simulink model "gtm_design"  (R2021b)
settings: Solver=VariableStepAuto  StartTime=0.0  StopTime=30  MinStep=0.0049  RelTol=1e-3
StopFcn:
  | MWSout=grabmws(bdroot);
  | MWSout.lastrun=datestr(now);
values from neighbouring files (symbols this model uses):
  g = 32.17405    [SingleDOF.m]    (also in layer1atm.m; mainSimple.m = 32.174; simio.m = [dx(Index.EOM(1:6)); delta(:)-f; -delta(:)-f ])
  GuidanceMode = 1    [mainSimple.m]    (also in setup.m)
  knots2fps = 1/fps2knots    (= 1.687800745)    [main.m]    (also in mainSimple.m = 1.68781)
  s = tf('s')    [SingleDOF.m]    (also in main.m; mainSimple.m; newmain.m)
undefined symbols (not defined in the file or in its folder): Aero, aftfuel, aftfuel_pos, AILL, AILLC, AILR, AILRC, alpha_deg, altitude_ft, Ax_g, Ay_g, Az_g, b, beta_deg, bias, BRAKEC, Cbar, cg_pos0, cg_shift_gear, DamageCase, DamageModels, DamageOnsetTime, Earth, ELLIB, ELLIBC, ELLOB, ELLOBC, ELRIB, ELRIBC, ELROB, ELROBC, engl_ang, engl_pos, engr_ang, engr_pos, FLAPLC, FLAPLIB, FLAPLOB, FLAPRC, FLAPRIB, FLAPROB, FuelUsed_Init, fwdfuel, fwdfuel_pos, GEAR, GEARC, Inertia0, Inertia_shift_gear, Ixx_model, Iyy_model, Izz_model, KTAS, LandingGear, LengON, LinearizeModeOn, m, MORPHLC, MORPHRC, NAV_altitude_m, NAV_latitude_deg ... (+51)
libraries: simulink_extras x39, simulink_need_slupdate x30, LPVBlockLibrary x9, aerolibconvert2 x7, simulink x3, aerolibtransform2 x3, UserContent_lib x2, uavalgslib x2, robotcorelib x1, uavutilslib x1
(part 5 of 7)

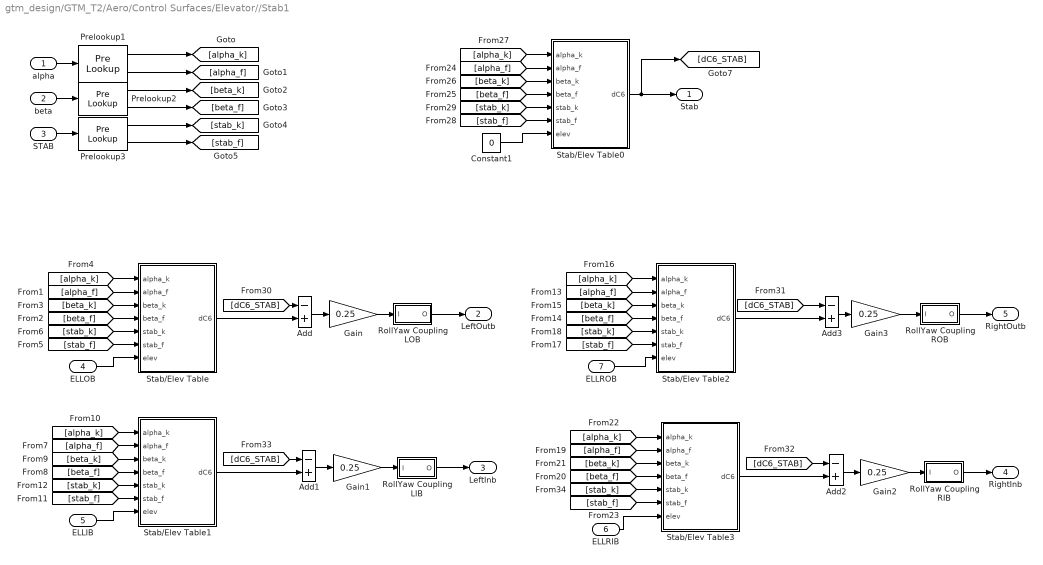
== system gtm_design/GTM_T2/Aero/Control Surfaces/Elevator//Stab1 ==
  alpha : Inport
  beta : Inport  Port=2
  STAB : Inport  Port=3
  ELLOB : Inport  Port=4
  ELLIB : Inport  Port=5
  ELLRIB : Inport  Port=6
  ELLROB : Inport  Port=7
  Add{,1..3} (4 alike) : Sum  Inputs=-+
  Constant1 : Constant  Value=0
  Gain{,1..3} (4 alike) : Gain  Gain=0.25
  Prelookup1 : PreLookup  BreakpointsData=Aero.dC3_ele.alpha  IndexSearchMethod=Linear search  BeginIndexSearchUsingPreviousIndexResult=on  ExtrapMethod=Linear
  Prelookup2 : PreLookup  BreakpointsData=Aero.dC3_ele.beta  IndexSearchMethod=Linear search  BeginIndexSearchUsingPreviousIndexResult=on  ExtrapMethod=Linear
  Prelookup3 : PreLookup  BreakpointsData=Aero.dC3_ele.stab  IndexSearchMethod=Linear search  BeginIndexSearchUsingPreviousIndexResult=on  ExtrapMethod=Linear
  RollYaw Coupling LIB : Subsystem  mask{arm=-0.03}
      mask prompts: arm "Moment arm (nd)"
      mask help:
      | Approximates roll/yaw coupling of split longitudinal surface
      | deflections (spoilers, elevators, flaps) where the base aero data only
      | has CX, CZ, and Cm. Input should be a 6 element vector of the aero
      | coefficients [CZ CY CZ Cl Cm Cn].
      |
      | Cl = Cl_input + arm*CZ_input
      | Cn = Cn_input + arm*CX_input
      mask init:
      | Kc = eye(6);
      | 
      | Kc(4,3) = arm; % Cl = Cl + arm*CZ
      | Kc(6,1) = -arm; % Cn = Cn - arm*CX
  RollYaw Coupling LOB : Subsystem  mask{arm=-0.07}
      mask prompts: arm "Moment arm (nd)"
      mask help:
      | Approximates roll/yaw coupling of split longitudinal surface
      | deflections (spoilers, elevators, flaps) where the base aero data only
      | has CX, CZ, and Cm. Input should be a 6 element vector of the aero
      | coefficients [CZ CY CZ Cl Cm Cn].
      |
      | Cl = Cl_input + arm*CZ_input
      | Cn = Cn_input + arm*CX_input
      mask init:
      | Kc = eye(6);
      | 
      | Kc(4,3) = arm; % Cl = Cl + arm*CZ
      | Kc(6,1) = -arm; % Cn = Cn - arm*CX
  RollYaw Coupling RIB : Subsystem  mask{arm=0.03}
      mask prompts: arm "Moment arm (nd)"
      mask help:
      | Approximates roll/yaw coupling of split longitudinal surface
      | deflections (spoilers, elevators, flaps) where the base aero data only
      | has CX, CZ, and Cm. Input should be a 6 element vector of the aero
      | coefficients [CZ CY CZ Cl Cm Cn].
      |
      | Cl = Cl_input + arm*CZ_input
      | Cn = Cn_input + arm*CX_input
      mask init:
      | Kc = eye(6);
      | 
      | Kc(4,3) = arm; % Cl = Cl + arm*CZ
      | Kc(6,1) = -arm; % Cn = Cn - arm*CX
  RollYaw Coupling ROB : Subsystem  mask{arm=0.07}
      mask prompts: arm "Moment arm (nd)"
      mask help:
      | Approximates roll/yaw coupling of split longitudinal surface
      | deflections (spoilers, elevators, flaps) where the base aero data only
      | has CX, CZ, and Cm. Input should be a 6 element vector of the aero
      | coefficients [CZ CY CZ Cl Cm Cn].
      |
      | Cl = Cl_input + arm*CZ_input
      | Cn = Cn_input + arm*CX_input
      mask init:
      | Kc = eye(6);
      | 
      | Kc(4,3) = arm; % Cl = Cl + arm*CZ
      | Kc(6,1) = -arm; % Cn = Cn - arm*CX
  Stab/Elev Table : Subsystem
  Stab/Elev Table0 : Subsystem
  Stab/Elev Table1 : Subsystem
  Stab/Elev Table2 : Subsystem
  Stab/Elev Table3 : Subsystem
  Stab : Outport
  LeftOutb : Outport  Port=2
  LeftInb : Outport  Port=3
  RightInb : Outport  Port=4
  RightOutb : Outport  Port=5
  wires:
  RollYaw Coupling RIB/1(O) -> RightInb/1
  RollYaw Coupling ROB/1(O) -> RightOutb/1
  RollYaw Coupling LIB/1(O) -> LeftInb/1
  RollYaw Coupling LOB/1(O) -> LeftOutb/1
  Stab/Elev Table0/1(dC6) -> [dC6_STAB], Stab/1
  [dC6_STAB] -> Add1/1
  Stab/Elev Table3/1(dC6) -> Add2/2
  [dC6_STAB] -> Add2/1
  [dC6_STAB] -> Add3/1
  Stab/Elev Table2/1(dC6) -> Add3/2
  Stab/Elev Table1/1(dC6) -> Add1/2
  Constant1/1 -> Stab/Elev Table0/7(elev)
  [stab_f] -> Stab/Elev Table0/6(stab_f)
  [stab_k] -> Stab/Elev Table0/5(stab_k)
  [beta_f] -> Stab/Elev Table0/4(beta_f)
  [beta_k] -> Stab/Elev Table0/3(beta_k)
  [alpha_f] -> Stab/Elev Table0/2(alpha_f)
  [alpha_k] -> Stab/Elev Table0/1(alpha_k)
  [dC6_STAB] -> Add/1
  Stab/Elev Table/1(dC6) -> Add/2
  ELLRIB/1 -> Stab/Elev Table3/7(elev)
  [stab_f] -> Stab/Elev Table3/6(stab_f)
  [stab_k] -> Stab/Elev Table3/5(stab_k)
  [beta_f] -> Stab/Elev Table3/4(beta_f)
  [beta_k] -> Stab/Elev Table3/3(beta_k)
  [alpha_f] -> Stab/Elev Table3/2(alpha_f)
  [alpha_k] -> Stab/Elev Table3/1(alpha_k)
  ELLROB/1 -> Stab/Elev Table2/7(elev)
  [stab_f] -> Stab/Elev Table2/6(stab_f)
  [stab_k] -> Stab/Elev Table2/5(stab_k)
  [beta_f] -> Stab/Elev Table2/4(beta_f)
  [beta_k] -> Stab/Elev Table2/3(beta_k)
  [alpha_f] -> Stab/Elev Table2/2(alpha_f)
  [alpha_k] -> Stab/Elev Table2/1(alpha_k)
  ELLIB/1 -> Stab/Elev Table1/7(elev)
  [stab_f] -> Stab/Elev Table1/6(stab_f)
  [stab_k] -> Stab/Elev Table1/5(stab_k)
  [beta_f] -> Stab/Elev Table1/4(beta_f)
  [beta_k] -> Stab/Elev Table1/3(beta_k)
  [alpha_f] -> Stab/Elev Table1/2(alpha_f)
  [alpha_k] -> Stab/Elev Table1/1(alpha_k)
  ELLOB/1 -> Stab/Elev Table/7(elev)
  [stab_f] -> Stab/Elev Table/6(stab_f)
  [stab_k] -> Stab/Elev Table/5(stab_k)
  [beta_f] -> Stab/Elev Table/4(beta_f)
  [beta_k] -> Stab/Elev Table/3(beta_k)
  [alpha_f] -> Stab/Elev Table/2(alpha_f)
  [alpha_k] -> Stab/Elev Table/1(alpha_k)
  Add3/1 -> Gain3/1
  Add2/1 -> Gain2/1
  Add1/1 -> Gain1/1
  Add/1 -> Gain/1
  Gain3/1 -> RollYaw Coupling ROB/1(I)
  Gain2/1 -> RollYaw Coupling RIB/1(I)
  Gain1/1 -> RollYaw Coupling LIB/1(I)
  Gain/1 -> RollYaw Coupling LOB/1(I)
  Prelookup3/2 -> [stab_f]
  Prelookup3/1 -> [stab_k]
  Prelookup2/2 -> [beta_f]
  Prelookup2/1 -> [beta_k]
  Prelookup1/2 -> [alpha_f]
  Prelookup1/1 -> [alpha_k]
  STAB/1 -> Prelookup3/1
  beta/1 -> Prelookup2/1
  alpha/1 -> Prelookup1/1

== system gtm_design/GTM_T2/Aero/Control Surfaces/Flaps ==
  alpha : Inport
  beta : Inport  Port=2
  FLAPLIB : Inport  Port=3
  MORPHL : Inport  Port=4
  FLAPRIB : Inport  Port=5
  MORPHR : Inport  Port=6
  Gain10 : Gain  Gain=Aero.flaps.flaprib
  Gain11 : Gain  Gain=Aero.flaps.flaprob
  Gain8 : Gain  Gain=Aero.flaps.flaplob
  Gain9 : Gain  Gain=Aero.flaps.flaplib
  Subsystem : Subsystem
  Sum : Sum  Inputs=|++
  Sum1 : Sum  Inputs=|++
  LeftMorph : Outport
  LeftFlap : Outport  Port=2
  RightFlap : Outport  Port=3
  RightMorph : Outport  Port=4
  wires:
  FLAPRIB/1 -> Gain11/1, Gain10/1
  FLAPLIB/1 -> Gain8/1, Gain9/1
  Gain9/1 -> Sum/1
  alpha/1 -> Subsystem/1(alpha)
  beta/1 -> Subsystem/2(beta)
  Gain8/1 -> Sum/2
  Gain10/1 -> Sum1/1
  Gain11/1 -> Sum1/2
  Sum/1 -> LeftFlap/1
  Sum1/1 -> RightFlap/1
  Subsystem/1(LeftOutb) -> LeftMorph/1
  Subsystem/2(RightOutb) -> RightMorph/1
  MORPHL/1 -> Subsystem/3(MORPHL)
  MORPHR/1 -> Subsystem/4(MORPHR)

== system gtm_design/GTM_T2/Aero/Control Surfaces/Gear ==
  alpha : Inport
  gear : Inport  Port=2
  Assignment to Longitudinal : Assignment  IndexMode=Zero-based  IndexOptions=Index vector (dialog)  Indices=[0 2 4]  OutputSizes=[1 1]
  Compare To Zero : simulink/Logic and Bit Operations/Compare To Zero  relop=~=  OutDataTypeStr=uint8  ZeroCross=off
  Constant : Constant  Value=zeros(6,1)
  Constant2 : Constant  Value=[0:2]  OutDataTypeStr=uint32
  Data Type Conversion2 : DataTypeConversion  OutDataTypeStr=uint32
  PreLookup Index Search1 : simulink_need_slupdate/PreLookup Index Search  bpData=Aero.dC3_lgr.alpha  searchMode=Binary Search  cacheBpFlag=on  outputFlag=off  IndexDataType=uint32  extrapMode=Linear Extrapolation  rangeErrorMode=None
      settings: SourceProductBaseCode=SL
  TableLookup : simulink_need_slupdate/Interpolation (n-D) using PreLookup  numDimsPopupSelect=3  explicitNumDims=2  table=Aero.dC3_lgr.data  interpMethod=Linear  extrapMethod=Linear  rangeErrorMode=None  NumSelectionDims=2
      settings: SourceProductBaseCode=SL
  LandingGear : Outport
  wires:
  gear/1 -> Compare To Zero/1
  Compare To Zero/1 -> Data Type Conversion2/1
  alpha/1 -> PreLookup Index Search1/1
  PreLookup Index Search1/1 -> TableLookup/1
  Constant2/1 -> TableLookup/3
  TableLookup/1 -> Assignment to Longitudinal/2
  Constant/1 -> Assignment to Longitudinal/1
  Assignment to Longitudinal/1 -> LandingGear/1
  Data Type Conversion2/1 -> TableLookup/2

== system gtm_design/GTM_T2/Aero/Control Surfaces/Implement Damage Models ==
  SurfVec : Inport
  damagecase : Inport  Port=2
  Implement Damage Models : MATLAB Function  TreatAsAtomicUnit=on
  Reshape : Reshape
  dC6 : Outport
  wires:
  Reshape/1 -> dC6/1
  damagecase/1 -> Implement Damage Models/2(DamageCase)
  Implement Damage Models/1(dC6) -> Reshape/1
  SurfVec/1 -> Implement Damage Models/1(SurfVec)

== system gtm_design/GTM_T2/Aero/Control Surfaces/Rudder ==
  alpha : Inport
  beta : Inport  Port=2
  RUDU : Inport  Port=3
  RUDL : Inport  Port=4
  Gains : Subsystem  mask{gains=[0.5  0.5  0.5  0.67  0.67  0.5]}
      mask prompts: gains "Mask Parameter 1:"
      mask help: Gains for each aerodynamic coefficient.
      mask Display: disp(['[' num2str(gains) ']'])
  Gains1 : Subsystem  mask{gains=[0.5  0.5  0.5  0.33  0.33  0.5]}
      mask prompts: gains "Mask Parameter 1:"
      mask help: Gains for each aerodynamic coefficient.
      mask Display: disp(['[' num2str(gains) ']'])
  Lower Rudder : Subsystem
  Upper Rudder : Subsystem
  Upper : Outport
  Lower : Outport  Port=2
  wires:
  RUDL/1 -> Lower Rudder/3(rud)
  Gains1/1(dC6) -> Lower/1
  RUDU/1 -> Upper Rudder/3(rud)
  beta/1 -> Lower Rudder/2(beta), Upper Rudder/2(beta)
  Gains/1(dC6) -> Upper/1
  alpha/1 -> Lower Rudder/1(alpha), Upper Rudder/1(alpha)
  Upper Rudder/1(dC6) -> Gains/1(dC6_in)
  Lower Rudder/1(dC6) -> Gains1/1(dC6_in)

== system gtm_design/GTM_T2/Aero/Control Surfaces/Spoilers ==
  alpha : Inport
  beta : Inport  Port=2
  SPLLIB : Inport  Port=3
  SPLRIB : Inport  Port=4
  SPLLOB : Inport  Port=5
  SPLROB : Inport  Port=6
  Gains1 : Subsystem  mask{gains=|}
      mask gains=|
      | [0.45	0.45	0.45	0.26	0.45	0.26
      | ]
      mask prompts: gains "Mask Parameter 1:"
      mask help: Gains for each aerodynamic coefficient.
      mask Display: disp(['[' num2str(gains) ']'])
  Gains2 : Subsystem  mask{gains=|}
      mask gains=|
      | [0.45	0.45	0.45	0.26	0.45	0.26
      | ]
      mask prompts: gains "Mask Parameter 1:"
      mask help: Gains for each aerodynamic coefficient.
      mask Display: disp(['[' num2str(gains) ']'])
  Gains3 : Subsystem  mask{gains=|}
      mask gains=|
      | [0.55	0.55	0.55	0.74	0.55	0.74
      | ]
      mask prompts: gains "Mask Parameter 1:"
      mask help: Gains for each aerodynamic coefficient.
      mask Display: disp(['[' num2str(gains) ']'])
  Gains4 : Subsystem  mask{gains=|}
      mask gains=|
      | [0.55	0.55	0.55	0.74	0.55	0.74
      | ]
      mask prompts: gains "Mask Parameter 1:"
      mask help: Gains for each aerodynamic coefficient.
      mask Display: disp(['[' num2str(gains) ']'])
  InboardSpoilers : Subsystem
  OutboardSpoilers : Subsystem
  LeftInb : Outport
  LeftOutb : Outport  Port=2
  RightInb : Outport  Port=3
  RightOutb : Outport  Port=4
  wires:
  OutboardSpoilers/2(Right) -> Gains4/1(dC6_in)
  InboardSpoilers/2(Right) -> Gains1/1(dC6_in)
  SPLROB/1 -> OutboardSpoilers/4(SPLRIB)
  SPLLOB/1 -> OutboardSpoilers/3(SPLLIB)
  SPLRIB/1 -> InboardSpoilers/4(SPLRIB)
  SPLLIB/1 -> InboardSpoilers/3(SPLLIB)
  beta/1 -> OutboardSpoilers/2(beta), InboardSpoilers/2(beta)
  alpha/1 -> OutboardSpoilers/1(alpha), InboardSpoilers/1(alpha)
  OutboardSpoilers/1(Left) -> Gains3/1(dC6_in)
  InboardSpoilers/1(Left) -> Gains2/1(dC6_in)
  Gains2/1(dC6) -> LeftInb/1
  Gains1/1(dC6) -> RightInb/1
  Gains3/1(dC6) -> LeftOutb/1
  Gains4/1(dC6) -> RightOutb/1

== system gtm_design/GTM_T2/Aero/Dynamic Derviatives/Forced Oscillation with Damage Increments ==
  alpha : Inport
  TAS : Inport  Port=2
  pqr : Inport  Port=3
  AC_Params : Inport  Port=4
  DamageCase : Inport  Port=5
  Action Port : ActionPort  ActionPortLabel=case [ 1 2 3 4 5 6 ]:
  Add : Sum  Inputs=+++
  Add1 : Sum
  Assignment to CY : Assignment  IndexMode=Zero-based  IndexOptions=Index vector (dialog)  Indices=1  OutputSizes=[1 1]
  Constant4 : Constant  Value=zeros(6,1)
  Damage Effects-Increments : Subsystem
  Damage Effects-Scaling : Subsystem
  Forced Oscillation : Subsystem
  Normalize : Subsystem
  Product1 : Product  RndMeth=Zero
  Product2 : Product  RndMeth=Zero
  Product3 : Product  RndMeth=Zero
  dC6 : Outport
  wires:
  Assignment to CY/1 -> Add1/1
  Add/1 -> Add1/2
  Product2/1 -> Add/1
  Product1/1 -> Add/2
  Product3/1 -> Add/3
  Forced Oscillation/3(dC6_r) -> Product3/2
  Forced Oscillation/2(dC6_q) -> Product1/2
  Forced Oscillation/1(dC6_p) -> Product2/2
  Normalize/1(pqrhat) -> Damage Effects-Increments/2(pqr), Forced Oscillation/2(pqr)
  AC_Params/1 -> Normalize/3(AC_Params)
  TAS/1 -> Normalize/2(TAS)
  pqr/1 -> Normalize/1(pqr)
  Add1/1 -> dC6/1
  Constant4/1 -> Assignment to CY/1
  Damage Effects-Increments/1(Increment) -> Assignment to CY/2
  Damage Effects-Scaling/3(Scaling_p) -> Product2/1
  Damage Effects-Scaling/2(Scaling_q) -> Product1/1
  Damage Effects-Scaling/1(Scaling_r) -> Product3/1
  DamageCase/1 -> Damage Effects-Increments/3(DamageCase), Damage Effects-Scaling/2(DamageCase)
  alpha/1 -> Damage Effects-Increments/1(alpha), Damage Effects-Scaling/1(alpha), Forced Oscillation/1(alpha)

== system gtm_design/GTM_T2/Aero/Dynamic Derviatives/Rotary Blended UnDamaged Case ==
  alpha : Inport
  beta : Inport  Port=2
  TAS : Inport  Port=3
  pqr : Inport  Port=4
  AC_Params : Inport  Port=5
  Action Port : ActionPort  ActionPortLabel=default:
  Add : Sum  Inputs=++++
  Blending Function : MATLAB Function  TreatAsAtomicUnit=on
  Bus Selector2 : BusSelector  OutputSignals=B,Cbar
  Forced Oscillation : Subsystem
  Rotary Balance : Subsystem
  Saturation : Saturate
  Saturation1 : Saturate  UpperLimit=10000  LowerLimit=1
  dC6 : Outport
  wires:
  Forced Oscillation/3(dC6_r) -> Add/4
  Forced Oscillation/2(dC6_q) -> Add/3
  Forced Oscillation/1(dC6_p) -> Add/2
  Rotary Balance/1(dC6) -> Add/1
  Add/1 -> dC6/1
  Bus Selector2/2 -> Blending Function/6(Cbar)  "<Cbar>"
  pqr/1 -> Blending Function/4(pqr)
  Saturation1/1 -> Blending Function/3(tas)
  Saturation/1 -> Rotary Balance/3(w)
  [alpha] -> Forced Oscillation/1(alpha)
  [beta] -> Rotary Balance/2(beta)
  [alpha] -> Rotary Balance/1(alpha)
  [beta] -> Blending Function/2(beta)
  beta/1 -> [beta]
  alpha/1 -> [alpha]
  [alpha] -> Blending Function/1(alpha)
  AC_Params/1 -> Bus Selector2/1
  TAS/1 -> Saturation1/1
  Bus Selector2/1 -> Blending Function/5(B)  "<B>"
  Blending Function/2(pqr_osc) -> Forced Oscillation/2(pqr)
  Blending Function/1(omega) -> Saturation/1

== system gtm_design/GTM_T2/AuxiliaryVariables/Atmos76/Atmos List ==
  I : Inport
  BusCreator : BusCreator  Inputs=7
  Demux2 : Demux  Outputs=6
      settings: DisplayOption=none
  Divide : Product  Inputs=*/
  Standard Temp. K : Constant  Value=288.15
  O : Outport
  wires:
  Divide/1 -> BusCreator/7  "tratio"
  Standard Temp. K/1 -> Divide/2
  BusCreator/1 -> O/1
  I/1 -> Demux2/1
  Demux2/1 -> BusCreator/1  "rho"
  Demux2/2 -> BusCreator/2  "pressure"
  Demux2/3 -> Divide/1, BusCreator/3  "temperature"
  Demux2/4 -> BusCreator/4  "cs"
  Demux2/5 -> BusCreator/5  "pratio"
  Demux2/6 -> BusCreator/6  "sqrsig"

== system gtm_design/GTM_T2/AuxiliaryVariables/WindShear and Xform/WindShear ==
  note: ShearFactor = ln(h/.15) / ln(h/20), as per MIL-Spec: MIL-F-8785C
  In : Inport
  Constant2 : Constant  Value=log(20/.15);
  Divide : Product  Inputs=*/
  Gain : Gain  Gain=1/.15; %MILSpec constant
  Gain2 : Gain  Gain=1/1.8; % Scale to get unity gain@1000ft (instead of 20 ft)
  Math Function : Math  Operator=log  SignedPower=on  SaturateOnIntegerOverflow=on
  Saturation : Saturate  UpperLimit=1000  LowerLimit=1
  Out : Outport
  wires:
  Gain2/1 -> Out/1
  Saturation/1 -> Gain/1
  Divide/1 -> Gain2/1
  Constant2/1 -> Divide/2
  Math Function/1 -> Divide/1
  In/1 -> Saturation/1
  Gain/1 -> Math Function/1

== system gtm_design/GTM_T2/EOM/Aircraft 6DOF/3D Vector Cross Product ==
  A : Inport
  B : Inport  Port=2
  Demux : Demux  Outputs=3
      settings: DisplayOption=none
  Demux1 : Demux  Outputs=3
      settings: DisplayOption=none
  Gain : Gain  Gain=-1  SaturateOnIntegerOverflow=on  OutDataTypeStr=Inherit: Same as input  ParamDataTypeStr=Inherit: Same as input
  Ground : Ground
  Mux : Mux  Inputs=9
  Product : Product  Multiplication=Matrix(*)  SaturateOnIntegerOverflow=on  OutDataTypeStr=Inherit: Same as first input
  Reshape : Reshape  OutputDimensionality=Customize  OutputDimensions=[3,3]
  AxB : Outport
  wires:
  A/1 -> Demux/1, Gain/1
  Product/1 -> AxB/1
  Ground/1 -> Mux/1, Mux/5, Mux/9
  Gain/1 -> Demux1/1
  Demux/3 -> Mux/2
  Demux1/2 -> Mux/3
  Demux1/3 -> Mux/4
  Demux/1 -> Mux/6
  Demux/2 -> Mux/7
  Demux1/1 -> Mux/8
  Mux/1 -> Reshape/1
  Reshape/1 -> Product/1
  B/1 -> Product/2

== system gtm_design/GTM_T2/EOM/Aircraft 6DOF/3D Vector Cross Product1 ==
  A : Inport
  B : Inport  Port=2
  Demux : Demux  Outputs=3
      settings: DisplayOption=none
  Demux1 : Demux  Outputs=3
      settings: DisplayOption=none
  Gain : Gain  Gain=-1  SaturateOnIntegerOverflow=on  OutDataTypeStr=Inherit: Same as input  ParamDataTypeStr=Inherit: Same as input
  Ground : Ground
  Mux : Mux  Inputs=9
  Product : Product  Multiplication=Matrix(*)  SaturateOnIntegerOverflow=on  OutDataTypeStr=Inherit: Same as first input
  Reshape : Reshape  OutputDimensionality=Customize  OutputDimensions=[3,3]
  AxB : Outport
  wires:
  A/1 -> Demux/1, Gain/1
  Product/1 -> AxB/1
  Ground/1 -> Mux/1, Mux/5, Mux/9
  Gain/1 -> Demux1/1
  Demux/3 -> Mux/2
  Demux1/2 -> Mux/3
  Demux1/3 -> Mux/4
  Demux/1 -> Mux/6
  Demux/2 -> Mux/7
  Demux1/1 -> Mux/8
  Mux/1 -> Reshape/1
  Reshape/1 -> Product/1
  B/1 -> Product/2

== system gtm_design/GTM_T2/EOM/Aircraft 6DOF/Euler to DCM ==
  "Euler " : Inport
  Fcn : Fcn  Expr=u(4)*u(2)*u(6)+u(3)*u(1)
  Fcn1 : Fcn  Expr=u(3)*u(5)
  Fcn2 : Fcn  Expr=u(3)*u(2)*u(1)+u(6)*u(4)
  Fcn3 : Fcn  Expr=u(3)*u(2)*u(4)-u(6)*u(1)
  Fcn4 : Fcn  Expr=-u(2)
  Fcn5 : Fcn  Expr=u(5)*u(1)
  Fcn6 : Fcn  Expr=u(1)*u(2)*u(6)-u(3)*u(4)
  Fcn7 : Fcn  Expr=u(5)*u(6)
  Fcn8 : Fcn  Expr=u(5)*u(4)
  Mux : Mux  Inputs=2
  Mux1 : Mux  Inputs=9
  Reshape : Reshape  OutputDimensionality=Customize  OutputDimensions=[3,3]
  Trigonometric Function : Trigonometry
  Trigonometric Function1 : Trigonometry  Operator=cos
  DCM : Outport
  wires:
  "Euler "/1 -> Trigonometric Function1/1, Trigonometric Function/1
  Trigonometric Function/1 -> Mux/1
  Trigonometric Function1/1 -> Mux/2
  Mux/1 -> Fcn4/1, Fcn8/1, Fcn5/1, Fcn3/1, Fcn/1, Fcn7/1, Fcn6/1, Fcn1/1, Fcn2/1
  Mux1/1 -> Reshape/1
  Fcn7/1 -> Mux1/1
  Fcn6/1 -> Mux1/2
  Fcn/1 -> Mux1/3
  Fcn1/1 -> Mux1/4
  Fcn2/1 -> Mux1/5
  Fcn3/1 -> Mux1/6
  Fcn4/1 -> Mux1/7
  Fcn5/1 -> Mux1/8
  Fcn8/1 -> Mux1/9
  Reshape/1 -> DCM/1

== system gtm_design/GTM_T2/EOM/Aircraft 6DOF/Vlocal to LatLon ==
  I : Inport
  Constant1 : Constant  Value=-1
  "EarthRadius " : Constant  Value=Re
  Math Function1 : Math  Operator=reciprocal  SignedPower=on  SaturateOnIntegerOverflow=on
  Mux : Mux  Inputs=3
  Product : Product  Inputs=*/  RndMeth=Zero
  Selector : Selector  InputPortWidth=3  IndexOptions=Index vector (dialog)  Indices=3  OutputSizes=1
  Selector1 : Selector  InputPortWidth=3  IndexOptions=Index vector (dialog)  Indices=1  OutputSizes=1
  Sum2 : Sum  Inputs=|++
  Trigonometric Function : Trigonometry  Operator=cos
  O : Outport
  wires:
  "EarthRadius "/1 -> Sum2/2
  Sum2/1 -> Math Function1/1
  Trigonometric Function/1 -> Product/2
  Math Function1/1 -> Product/1, Mux/1
  Product/1 -> Mux/2
  Constant1/1 -> Mux/3
  Selector/1 -> Sum2/1
  I/1 -> Selector/1, Selector1/1
  Mux/1 -> O/1
  Selector1/1 -> Trigonometric Function/1

== system gtm_design/GTM_T2/EOM/Anti Windup/Subsystem1 ==
  I : Inport
  Constant1 : Constant  Value=2*pi
  Constant2 : Constant  Value=2*pi
  Constant3 : Constant  Value=2*pi
  Math Function1 : Math  Operator=rem  SignedPower=on  SaturateOnIntegerOverflow=on
  Sum : Sum  Inputs=|-+  SaturateOnIntegerOverflow=on
  Sum1 : Sum  Inputs=++|  SaturateOnIntegerOverflow=on
  Switch : Switch  Criteria=u2 > Threshold  Threshold=pi  SaturateOnIntegerOverflow=on
  Switch1 : Switch  SaturateOnIntegerOverflow=on
  Switch2 : Switch  Threshold=-pi  SaturateOnIntegerOverflow=on
  O : Outport
  wires:
  Switch1/1 -> O/1
  Switch/1 -> Switch1/1
  Switch2/1 -> Switch1/3
  Sum1/1 -> Switch2/3
  Constant3/1 -> Sum1/2
  Sum/1 -> Switch/1
  Constant2/1 -> Sum/1
  Math Function1/1 -> Switch1/2, Sum1/1, Switch2/2, Switch2/1, Switch/3, Sum/2, Switch/2
  I/1 -> Math Function1/1
  Constant1/1 -> Math Function1/2

== system gtm_design/GTM_T2/EOM/Anti Windup/Subsystem3 ==
  I : Inport
  Constant1 : Constant  Value=2*pi
  Constant2 : Constant  Value=2*pi
  Constant3 : Constant  Value=2*pi
  Math Function1 : Math  Operator=rem  SignedPower=on  SaturateOnIntegerOverflow=on
  Sum : Sum  Inputs=|-+  SaturateOnIntegerOverflow=on
  Sum1 : Sum  Inputs=++|  SaturateOnIntegerOverflow=on
  Switch : Switch  Criteria=u2 > Threshold  Threshold=pi  SaturateOnIntegerOverflow=on
  Switch1 : Switch  SaturateOnIntegerOverflow=on
  Switch2 : Switch  Threshold=-pi  SaturateOnIntegerOverflow=on
  O : Outport
  wires:
  Switch1/1 -> O/1
  Switch/1 -> Switch1/1
  Switch2/1 -> Switch1/3
  Sum1/1 -> Switch2/3
  Constant3/1 -> Sum1/2
  Sum/1 -> Switch/1
  Constant2/1 -> Sum/1
  Math Function1/1 -> Switch1/2, Sum1/1, Switch2/2, Switch2/1, Switch/3, Sum/2, Switch/2
  I/1 -> Math Function1/1
  Constant1/1 -> Math Function1/2

== system gtm_design/GTM_T2/EOM/Anti Windup/Subsystem4 ==
  I : Inport
  Constant1 : Constant  Value=2*pi
  Math Function1 : Math  Operator=rem  SignedPower=on  SaturateOnIntegerOverflow=on
  Math Function2 : Math  Operator=rem  SignedPower=on  SaturateOnIntegerOverflow=on
  Sum2 : Sum  Inputs=|++  SaturateOnIntegerOverflow=on
  O : Outport
  wires:
  Constant1/1 -> Math Function1/2, Math Function2/2, Sum2/2
  I/1 -> Math Function1/1
  Sum2/1 -> Math Function2/1
  Math Function1/1 -> Sum2/1
  Math Function2/1 -> O/1

== system gtm_design/GTM_T2/Engines/CG torque/3D Vector Cross Product ==
  A : Inport
  B : Inport  Port=2
  Demux : Demux  Outputs=3
      settings: DisplayOption=none
  Demux1 : Demux  Outputs=3
      settings: DisplayOption=none
  Gain : Gain  Gain=-1  SaturateOnIntegerOverflow=on  OutDataTypeStr=Inherit: Same as input  ParamDataTypeStr=Inherit: Same as input
  Ground : Ground
  Mux : Mux  Inputs=9
  Product : Product  Multiplication=Matrix(*)  SaturateOnIntegerOverflow=on  OutDataTypeStr=Inherit: Same as first input
  Reshape : Reshape  OutputDimensionality=Customize  OutputDimensions=[3,3]
  AxB : Outport
  wires:
  A/1 -> Demux/1, Gain/1
  Product/1 -> AxB/1
  Ground/1 -> Mux/1, Mux/5, Mux/9
  Gain/1 -> Demux1/1
  Demux/3 -> Mux/2
  Demux1/2 -> Mux/3
  Demux1/3 -> Mux/4
  Demux/1 -> Mux/6
  Demux/2 -> Mux/7
  Demux1/1 -> Mux/8
  Mux/1 -> Reshape/1
  Reshape/1 -> Product/1
  B/1 -> Product/2

== system gtm_design/GTM_T2/Engines/CG torque/3D Vector Cross Product1 ==
  A : Inport
  B : Inport  Port=2
  Demux : Demux  Outputs=3
      settings: DisplayOption=none
  Demux1 : Demux  Outputs=3
      settings: DisplayOption=none
  Gain : Gain  Gain=-1  SaturateOnIntegerOverflow=on  OutDataTypeStr=Inherit: Same as input  ParamDataTypeStr=Inherit: Same as input
  Ground : Ground
  Mux : Mux  Inputs=9
  Product : Product  Multiplication=Matrix(*)  SaturateOnIntegerOverflow=on  OutDataTypeStr=Inherit: Same as first input
  Reshape : Reshape  OutputDimensionality=Customize  OutputDimensions=[3,3]
  AxB : Outport
  wires:
  A/1 -> Demux/1, Gain/1
  Product/1 -> AxB/1
  Ground/1 -> Mux/1, Mux/5, Mux/9
  Gain/1 -> Demux1/1
  Demux/3 -> Mux/2
  Demux1/2 -> Mux/3
  Demux1/3 -> Mux/4
  Demux/1 -> Mux/6
  Demux/2 -> Mux/7
  Demux1/1 -> Mux/8
  Mux/1 -> Reshape/1
  Reshape/1 -> Product/1
  B/1 -> Product/2

== system gtm_design/GTM_T2/Engines/Left_Engine Jetcat P70/Throttle Lag1 ==
  throttle : Inport
  Gain : Gain  Gain=B  Multiplication=Matrix(K*u)
  Gain1 : Gain  Gain=A  Multiplication=Matrix(K*u)
  Gain2 : Gain  Gain=C  Multiplication=Matrix(K*u)
  Gain3 : Gain  Gain=flipud(B)/C(2)
  Integrator : Integrator  InitialConditionSource=external
  Sum1 : Sum  Inputs=|++
  y : Outport
  wires:
  Sum1/1 -> Integrator/1  "xdot"
  Gain1/1 -> Sum1/2
  Integrator/1 -> Gain1/1, Gain2/1
  Gain/1 -> Sum1/1
  Gain2/1 -> y/1
  throttle/1 -> Gain/1, Gain3/1
  Gain3/1 -> Integrator/2

== system gtm_design/GTM_T2/Engines/Right_Engine Jetcat P70/Throttle Lag1 ==
  throttle : Inport
  Gain : Gain  Gain=B  Multiplication=Matrix(K*u)
  Gain1 : Gain  Gain=A  Multiplication=Matrix(K*u)
  Gain2 : Gain  Gain=C  Multiplication=Matrix(K*u)
  Gain3 : Gain  Gain=flipud(B)/C(2)
  Integrator : Integrator  InitialConditionSource=external
  Sum1 : Sum  Inputs=|++
  y : Outport
  wires:
  Sum1/1 -> Integrator/1  "xdot"
  Gain1/1 -> Sum1/2
  Integrator/1 -> Gain1/1, Gain2/1
  Gain/1 -> Sum1/1
  Gain2/1 -> y/1
  throttle/1 -> Gain/1, Gain3/1
  Gain3/1 -> Integrator/2

== system gtm_design/GTM_T2/Landing Gear/LandingGear/Euler to DCM1 ==
  "Euler " : Inport
  Fcn : Fcn  Expr=u(4)*u(2)*u(6)+u(3)*u(1)
  Fcn1 : Fcn  Expr=u(3)*u(5)
  Fcn2 : Fcn  Expr=u(3)*u(2)*u(1)+u(6)*u(4)
  Fcn3 : Fcn  Expr=u(3)*u(2)*u(4)-u(6)*u(1)
  Fcn4 : Fcn  Expr=-u(2)
  Fcn5 : Fcn  Expr=u(5)*u(1)
  Fcn6 : Fcn  Expr=u(1)*u(2)*u(6)-u(3)*u(4)
  Fcn7 : Fcn  Expr=u(5)*u(6)
  Fcn8 : Fcn  Expr=u(5)*u(4)
  Mux : Mux  Inputs=2
  Mux1 : Mux  Inputs=9
  Reshape : Reshape  OutputDimensionality=Customize  OutputDimensions=[3,3]
  Trigonometric Function : Trigonometry
  Trigonometric Function1 : Trigonometry  Operator=cos
  DCM : Outport
  wires:
  "Euler "/1 -> Trigonometric Function1/1, Trigonometric Function/1
  Trigonometric Function/1 -> Mux/1
  Trigonometric Function1/1 -> Mux/2
  Mux/1 -> Fcn/1, Fcn7/1, Fcn6/1, Fcn1/1, Fcn2/1, Fcn4/1, Fcn8/1, Fcn5/1, Fcn3/1
  Mux1/1 -> Reshape/1
  Fcn7/1 -> Mux1/1
  Fcn6/1 -> Mux1/2
  Fcn/1 -> Mux1/3
  Fcn1/1 -> Mux1/4
  Fcn2/1 -> Mux1/5
  Fcn3/1 -> Mux1/6
  Fcn4/1 -> Mux1/7
  Fcn5/1 -> Mux1/8
  Fcn8/1 -> Mux1/9
  Reshape/1 -> DCM/1

== system gtm_design/GTM_T2/Landing Gear/LandingGear/Subsystem ==
  Alt : Inport
  Mux : Mux  Inputs=2
  Sum : Sum  Inputs=|+-
  Wheel Positions3 : Constant  Value=RunwayAlt
  Wheel Positions4 : Constant  Value=[0;0]
  cg_wrt_rwy : Outport
  wires:
  Mux/1 -> cg_wrt_rwy/1
  Sum/1 -> Mux/2
  Alt/1 -> Sum/1
  Wheel Positions4/1 -> Mux/1
  Wheel Positions3/1 -> Sum/2

== system gtm_design/GTM_T2/Sensors/Air Data/First Order Filter ==
  In : Inport
  Constant : Constant  Value=Timestep
  Constant1 : Constant  Value=tau
  Enabled Subsystem : Subsystem  TreatAsAtomicUnit=on
  Relational Operator : RelationalOperator  Operator=>  OutDataTypeStr=boolean  RndMeth=Nearest
  Switch : Switch  Threshold=0.5
  Out : Outport
  wires:
  Constant1/1 -> Enabled Subsystem/2(tau), Relational Operator/1
  Enabled Subsystem/1(Out) -> Switch/1
  Switch/1 -> Out/1
  In/1 -> Enabled Subsystem/1(In), Switch/3
  Relational Operator/1 -> Enabled Subsystem/Enable, Switch/2
  Constant/1 -> Relational Operator/2

== system gtm_design/GTM_T2/Sensors/Air Data/Sensor Model1 ==
  In1 : Inport
  Add : Sum  Inputs=+++
  Gain : Gain  Gain=scf
  Gear1 : Constant  Value=bias
  Gear2 : Constant  Value=noise_on
  Noise_on : Switch  Threshold=0.5  SaturateOnIntegerOverflow=on  InputSameDT=on
  White Noise : RandomNumber  Variance=sigma*sigma  Seed=round(seed*rand(1))  SampleTime=Timestep
  Out1 : Outport
  wires:
  Noise_on/1 -> Out1/1
  Gear2/1 -> Noise_on/2
  White Noise/1 -> Add/1
  Add/1 -> Noise_on/1
  Gear1/1 -> Add/2
  Gain/1 -> Add/3
  In1/1 -> Noise_on/3, Gain/1

== system gtm_design/GTM_T2/Sensors/Air Data/Sensor Model2 ==
  In1 : Inport
  Add : Sum  Inputs=+++
  Gain : Gain  Gain=scf
  Gear1 : Constant  Value=bias
  Gear2 : Constant  Value=noise_on
  Noise_on : Switch  Threshold=0.5  SaturateOnIntegerOverflow=on  InputSameDT=on
  White Noise : RandomNumber  Variance=sigma*sigma  Seed=round(seed*rand(1))  SampleTime=Timestep
  Out1 : Outport
  wires:
  Noise_on/1 -> Out1/1
  Gear2/1 -> Noise_on/2
  White Noise/1 -> Add/1
  Add/1 -> Noise_on/1
  Gear1/1 -> Add/2
  Gain/1 -> Add/3
  In1/1 -> Noise_on/3, Gain/1

== system gtm_design/GTM_T2/Sensors/Air Data/Sensor Model3 ==
  In1 : Inport
  Add : Sum  Inputs=+++
  Gain : Gain  Gain=scf
  Gear1 : Constant  Value=bias
  Gear2 : Constant  Value=noise_on
  Noise_on : Switch  Threshold=0.5  SaturateOnIntegerOverflow=on  InputSameDT=on
  White Noise : RandomNumber  Variance=sigma*sigma  Seed=round(seed*rand(1))  SampleTime=Timestep
  Out1 : Outport
  wires:
  Noise_on/1 -> Out1/1
  Gear2/1 -> Noise_on/2
  White Noise/1 -> Add/1
  Add/1 -> Noise_on/1
  Gear1/1 -> Add/2
  Gain/1 -> Add/3
  In1/1 -> Noise_on/3, Gain/1

== system gtm_design/GTM_T2/Sensors/Air Data/Sensor Model4 ==
  In1 : Inport
  Add : Sum  Inputs=+++
  Gain : Gain  Gain=scf
  Gear1 : Constant  Value=bias
  Gear2 : Constant  Value=noise_on
  Noise_on : Switch  Threshold=0.5  SaturateOnIntegerOverflow=on  InputSameDT=on
  White Noise : RandomNumber  Variance=sigma*sigma  Seed=round(seed*rand(1))  SampleTime=Timestep
  Out1 : Outport
  wires:
  Noise_on/1 -> Out1/1
  Gear2/1 -> Noise_on/2
  White Noise/1 -> Add/1
  Add/1 -> Noise_on/1
  Gear1/1 -> Add/2
  Gain/1 -> Add/3
  In1/1 -> Noise_on/3, Gain/1

== system gtm_design/GTM_T2/Sensors/Air Data/Sensor Model5 ==
  In1 : Inport
  Add : Sum  Inputs=+++
  Gain : Gain  Gain=scf
  Gear1 : Constant  Value=bias
  Gear2 : Constant  Value=noise_on
  Noise_on : Switch  Threshold=0.5  SaturateOnIntegerOverflow=on  InputSameDT=on
  White Noise : RandomNumber  Variance=sigma*sigma  Seed=round(seed*rand(1))  SampleTime=Timestep
  Out1 : Outport
  wires:
  Noise_on/1 -> Out1/1
  Gear2/1 -> Noise_on/2
  White Noise/1 -> Add/1
  Add/1 -> Noise_on/1
  Gear1/1 -> Add/2
  Gain/1 -> Add/3
  In1/1 -> Noise_on/3, Gain/1

== system gtm_design/GTM_T2/Sensors/Air Data/Sensor Model6 ==
  In1 : Inport
  Add : Sum  Inputs=+++
  Gain : Gain  Gain=scf
  Gear1 : Constant  Value=bias
  Gear2 : Constant  Value=noise_on
  Noise_on : Switch  Threshold=0.5  SaturateOnIntegerOverflow=on  InputSameDT=on
  White Noise : RandomNumber  Variance=sigma*sigma  Seed=round(seed*rand(1))  SampleTime=Timestep
  Out1 : Outport
  wires:
  Noise_on/1 -> Out1/1
  Gear2/1 -> Noise_on/2
  White Noise/1 -> Add/1
  Add/1 -> Noise_on/1
  Gear1/1 -> Add/2
  Gain/1 -> Add/3
  In1/1 -> Noise_on/3, Gain/1

== system gtm_design/GTM_T2/Sensors/MAG3 IMU/Sensor Model1 ==
  In1 : Inport
  Add : Sum  Inputs=+++
  Gain : Gain  Gain=scf
  Gear1 : Constant  Value=bias
  Gear2 : Constant  Value=noise_on
  Noise_on : Switch  Threshold=0.5  SaturateOnIntegerOverflow=on  InputSameDT=on
  White Noise : RandomNumber  Variance=sigma*sigma  Seed=round(seed*rand(1))  SampleTime=Timestep
  Out1 : Outport
  wires:
  Noise_on/1 -> Out1/1
  Gear2/1 -> Noise_on/2
  White Noise/1 -> Add/1
  Add/1 -> Noise_on/1
  Gear1/1 -> Add/2
  Gain/1 -> Add/3
  In1/1 -> Noise_on/3, Gain/1

== system gtm_design/GTM_T2/Sensors/MAG3 IMU/Sensor Model2 ==
  In1 : Inport
  Add : Sum  Inputs=+++
  Gain : Gain  Gain=scf
  Gear1 : Constant  Value=bias
  Gear2 : Constant  Value=noise_on
  Noise_on : Switch  Threshold=0.5  SaturateOnIntegerOverflow=on  InputSameDT=on
  White Noise : RandomNumber  Variance=sigma*sigma  Seed=round(seed*rand(1))  SampleTime=Timestep
  Out1 : Outport
  wires:
  Noise_on/1 -> Out1/1
  Gear2/1 -> Noise_on/2
  White Noise/1 -> Add/1
  Add/1 -> Noise_on/1
  Gear1/1 -> Add/2
  Gain/1 -> Add/3
  In1/1 -> Noise_on/3, Gain/1

== system gtm_design/GTM_T2/Sensors/MAG3 IMU/Sensor Model3 ==
  In1 : Inport
  Add : Sum  Inputs=+++
  Gain : Gain  Gain=scf
  Gear1 : Constant  Value=bias
  Gear2 : Constant  Value=noise_on
  Noise_on : Switch  Threshold=0.5  SaturateOnIntegerOverflow=on  InputSameDT=on
  White Noise : RandomNumber  Variance=sigma*sigma  Seed=round(seed*rand(1))  SampleTime=Timestep
  Out1 : Outport
  wires:
  Noise_on/1 -> Out1/1
  Gear2/1 -> Noise_on/2
  White Noise/1 -> Add/1
  Add/1 -> Noise_on/1
  Gear1/1 -> Add/2
  Gain/1 -> Add/3
  In1/1 -> Noise_on/3, Gain/1

== system gtm_design/GTM_T2/Sensors/MAG3 IMU/Sensor Model4 ==
  In1 : Inport
  Add : Sum  Inputs=+++
  Gain : Gain  Gain=scf
  Gear1 : Constant  Value=bias
  Gear2 : Constant  Value=noise_on
  Noise_on : Switch  Threshold=0.5  SaturateOnIntegerOverflow=on  InputSameDT=on
  White Noise : RandomNumber  Variance=sigma*sigma  Seed=round(seed*rand(1))  SampleTime=Timestep
  Out1 : Outport
  wires:
  Noise_on/1 -> Out1/1
  Gear2/1 -> Noise_on/2
  White Noise/1 -> Add/1
  Add/1 -> Noise_on/1
  Gear1/1 -> Add/2
  Gain/1 -> Add/3
  In1/1 -> Noise_on/3, Gain/1

== system gtm_design/GTM_T2/Sensors/MAG3 IMU/Sensor Model5 ==
  In1 : Inport
  Add : Sum  Inputs=+++
  Gain : Gain  Gain=scf
  Gear1 : Constant  Value=bias
  Gear2 : Constant  Value=noise_on
  Noise_on : Switch  Threshold=0.5  SaturateOnIntegerOverflow=on  InputSameDT=on
  White Noise : RandomNumber  Variance=sigma*sigma  Seed=round(seed*rand(1))  SampleTime=Timestep
  Out1 : Outport
  wires:
  Noise_on/1 -> Out1/1
  Gear2/1 -> Noise_on/2
  White Noise/1 -> Add/1
  Add/1 -> Noise_on/1
  Gear1/1 -> Add/2
  Gain/1 -> Add/3
  In1/1 -> Noise_on/3, Gain/1

== system gtm_design/GTM_T2/Sensors/MAG3 IMU/Sensor Model6 ==
  In1 : Inport
  Add : Sum  Inputs=+++
  Gain : Gain  Gain=scf
  Gear1 : Constant  Value=bias
  Gear2 : Constant  Value=noise_on
  Noise_on : Switch  Threshold=0.5  SaturateOnIntegerOverflow=on  InputSameDT=on
  White Noise : RandomNumber  Variance=sigma*sigma  Seed=round(seed*rand(1))  SampleTime=Timestep
  Out1 : Outport
  wires:
  Noise_on/1 -> Out1/1
  Gear2/1 -> Noise_on/2
  White Noise/1 -> Add/1
  Add/1 -> Noise_on/1
  Gear1/1 -> Add/2
  Gain/1 -> Add/3
  In1/1 -> Noise_on/3, Gain/1

== system gtm_design/GTM_T2/Sensors/MIDG II 50 Hz/MIDG Labels ==
  I : Inport
  Bus Creator : BusCreator  Inputs=9
  Demux : Demux  Outputs=9
  O : Outport
  wires:
  I/1 -> Demux/1
  Bus Creator/1 -> O/1
  Demux/2 -> Bus Creator/2  "theta_deg"
  Demux/3 -> Bus Creator/3  "psi_deg"
  Demux/1 -> Bus Creator/1  "phi_deg"
  Demux/4 -> Bus Creator/4  "NAV_latitude_deg"
  Demux/5 -> Bus Creator/5  "NAV_longitude_deg"
  Demux/6 -> Bus Creator/6  "NAV_altitude_m"
  Demux/7 -> Bus Creator/7  "NAV_Vn_mps"
  Demux/8 -> Bus Creator/8  "NAV_Ve_mps"
  Demux/9 -> Bus Creator/9  "NAV_Vu_mps"

== system gtm_design/GTM_T2/Sensors/MIDG II 50 Hz/Map+//-180 ==
  I : Inport
  Constant : Constant  Value=-360
  Constant1 : Constant  Value=0
  Sum : Sum  Inputs=|++
  if>180sub360 : Switch  Threshold=180
  O : Outport
  wires:
  if>180sub360/1 -> Sum/2
  Sum/1 -> O/1
  I/1 -> if>180sub360/2, Sum/1
  Constant1/1 -> if>180sub360/3
  Constant/1 -> if>180sub360/1

== system gtm_design/GTM_T2/Sensors/MIDG II 50 Hz/Sensor Model7 ==
  In1 : Inport
  Add : Sum  Inputs=+++
  Gain : Gain  Gain=scf
  Gear1 : Constant  Value=bias
  Gear2 : Constant  Value=noise_on
  Noise_on : Switch  Threshold=0.5  SaturateOnIntegerOverflow=on  InputSameDT=on
  White Noise : RandomNumber  Variance=sigma*sigma  Seed=round(seed*rand(1))  SampleTime=Timestep
  Out1 : Outport
  wires:
  Noise_on/1 -> Out1/1
  Gear2/1 -> Noise_on/2
  White Noise/1 -> Add/1
  Add/1 -> Noise_on/1
  Gear1/1 -> Add/2
  Gain/1 -> Add/3
  In1/1 -> Noise_on/3, Gain/1

== system gtm_design/GTM_T2/Sensors/MIDG II 50 Hz/Sensor Model8 ==
  In1 : Inport
  Add : Sum  Inputs=+++
  Gain : Gain  Gain=scf
  Gear1 : Constant  Value=bias
  Gear2 : Constant  Value=noise_on
  Noise_on : Switch  Threshold=0.5  SaturateOnIntegerOverflow=on  InputSameDT=on
  White Noise : RandomNumber  Variance=sigma*sigma  Seed=round(seed*rand(1))  SampleTime=Timestep
  Out1 : Outport
  wires:
  Noise_on/1 -> Out1/1
  Gear2/1 -> Noise_on/2
  White Noise/1 -> Add/1
  Add/1 -> Noise_on/1
  Gear1/1 -> Add/2
  Gain/1 -> Add/3
  In1/1 -> Noise_on/3, Gain/1

== system gtm_design/GTM_T2/Sensors/MIDG II 50 Hz/Sensor Model9 ==
  In1 : Inport
  Add : Sum  Inputs=+++
  Gain : Gain  Gain=scf
  Gear1 : Constant  Value=bias
  Gear2 : Constant  Value=noise_on
  Noise_on : Switch  Threshold=0.5  SaturateOnIntegerOverflow=on  InputSameDT=on
  White Noise : RandomNumber  Variance=sigma*sigma  Seed=round(seed*rand(1))  SampleTime=Timestep
  Out1 : Outport
  wires:
  Noise_on/1 -> Out1/1
  Gear2/1 -> Noise_on/2
  White Noise/1 -> Add/1
  Add/1 -> Noise_on/1
  Gear1/1 -> Add/2
  Gain/1 -> Add/3
  In1/1 -> Noise_on/3, Gain/1

== system gtm_design/GTM_T2/Sensors/MIDG II 50 Hz/TimeDelay with IC feedthrough ==
  I : Inport
  Clock : Clock
  Switch : Switch  Criteria=u2 > Threshold  Threshold=TimeDelay
  Transport Delay : TransportDelay  DelayTime=TimeDelay
      settings: AttributesFormatString=%<DelayTime>
  O : Outport
  wires:
  I/1 -> Transport Delay/1, Switch/3
  Clock/1 -> Switch/2
  Switch/1 -> O/1
  Transport Delay/1 -> Switch/1

== system gtm_design/GTM_T2/Sensors/Surface Pots/Sensor Model5 ==
  In1 : Inport
  Add : Sum  Inputs=+++
  Gain : Gain  Gain=scf
  Gear1 : Constant  Value=bias
  Gear2 : Constant  Value=noise_on
  Noise_on : Switch  Threshold=0.5  SaturateOnIntegerOverflow=on  InputSameDT=on
  White Noise : RandomNumber  Variance=sigma*sigma  Seed=round(seed*rand(1))  SampleTime=Timestep
  Out1 : Outport
  wires:
  Noise_on/1 -> Out1/1
  Gear2/1 -> Noise_on/2
  White Noise/1 -> Add/1
  Add/1 -> Noise_on/1
  Gear1/1 -> Add/2
  Gain/1 -> Add/3
  In1/1 -> Noise_on/3, Gain/1

== system gtm_design/GTM_T2/Sensors/Surface Pots/Surface Labels ==
  I : Inport
  Bus Creator : BusCreator  Inputs=12
  Demux : Demux  Outputs=12
  O : Outport
  wires:
  Bus Creator/1 -> O/1
  Demux/12 -> Bus Creator/12  "FLAPROB"
  Demux/11 -> Bus Creator/11  "FLAPRIB"
  Demux/10 -> Bus Creator/10  "FLAPLOB"
  Demux/9 -> Bus Creator/9  "FLAPLIB"
  Demux/8 -> Bus Creator/8  "RUDL"
  Demux/7 -> Bus Creator/7  "RUDU"
  Demux/6 -> Bus Creator/6  "AILR"
  Demux/5 -> Bus Creator/5  "AILL"
  Demux/4 -> Bus Creator/4  "ELRIB"
  Demux/3 -> Bus Creator/3  "ELROB"
  Demux/2 -> Bus Creator/2  "ELLIB"
  Demux/1 -> Bus Creator/1  "ELLOB"
  I/1 -> Demux/1

== system gtm_design/GTM_T2/TransportDelay/AntiAliasing/First Order Filter Continuous ==
  In : Inport
  Constant : Constant  Value=tau
  Divide : Product  Inputs=*/
  Integrator : Integrator  InitialConditionSource=external
  Sum : Sum  Inputs=-+|  InputSameDT=on  SaturateOnIntegerOverflow=on  OutDataTypeStr=Inherit: Same as first input
  Out : Outport
  wires:
  Constant/1 -> Divide/2
  Sum/1 -> Divide/1  "Error"
  In/1 -> Integrator/2, Sum/2
  Integrator/1 -> Out/1, Sum/1  "Y"
  Divide/1 -> Integrator/1  "Ydot"

== system gtm_design/GTM_T2/TransportDelay/Transport Delay on Bus/BusDelay ==
  In1 : Inport
  Bus Assignment : BusAssignment  AssignedSignals=alpha_deg,beta_deg,qbar_psf,KTAS,TEMPAMB_degF,altitude_ft
  Bus Selector1 : BusSelector  OutputSignals=alpha_deg,beta_deg,qbar_psf,KTAS,TEMPAMB_degF,altitude_ft  OutputAsBus=on
  Bus to Vector : BusToVector
  Demux : Demux  Outputs=6
  TimeDelay with IC feedthrough : Subsystem  mask{TimeDelay=15e-3}
      mask prompts: TimeDelay "Time Delay (sec)"
      mask help:
      | Implements Continuous Time Transport Delay with initial
      | outputs set to feedthrough with no delay.
      |
      |   output = input;   for t<TimeDelay
      |   output = input(t-tdelay); for t>=TimeDelay
  Out1 : Outport
  wires:
  In1/1 -> Bus Assignment/1, Bus Selector1/1
  Bus Selector1/1 -> Bus to Vector/1
  Bus to Vector/1 -> TimeDelay with IC feedthrough/1(I)
  TimeDelay with IC feedthrough/1(O) -> Demux/1
  Demux/1 -> Bus Assignment/2
  Demux/2 -> Bus Assignment/3
  Demux/3 -> Bus Assignment/4
  Demux/4 -> Bus Assignment/5
  Demux/5 -> Bus Assignment/6
  Demux/6 -> Bus Assignment/7
  Bus Assignment/1 -> Out1/1

== system gtm_design/GTM_T2/TransportDelay/Transport Delay on Bus/BusDelay1 ==
  In1 : Inport
  Bus Assignment : BusAssignment  AssignedSignals=phi_deg,theta_deg,psi_deg,NAV_latitude_deg,NAV_longitude_deg,NAV_altitude_m,NAV_Vn_mps,NAV_Ve_mps,NAV_Vu_mps
  Bus Selector1 : BusSelector  OutputSignals=phi_deg,theta_deg,psi_deg,NAV_latitude_deg,NAV_longitude_deg,NAV_altitude_m,NAV_Vn_mps,NAV_Ve_mps,NAV_Vu_mps  OutputAsBus=on
  Bus to Vector : BusToVector
  Demux : Demux  Outputs=9
  TimeDelay with IC feedthrough : Subsystem  mask{TimeDelay=15e-3}
      mask prompts: TimeDelay "Time Delay (sec)"
      mask help:
      | Implements Continuous Time Transport Delay with initial
      | outputs set to feedthrough with no delay.
      |
      |   output = input;   for t<TimeDelay
      |   output = input(t-tdelay); for t>=TimeDelay
  Out1 : Outport
  wires:
  In1/1 -> Bus Assignment/1, Bus Selector1/1
  Bus Selector1/1 -> Bus to Vector/1
  Bus to Vector/1 -> TimeDelay with IC feedthrough/1(I)
  TimeDelay with IC feedthrough/1(O) -> Demux/1
  Demux/1 -> Bus Assignment/2
  Demux/2 -> Bus Assignment/3
  Demux/3 -> Bus Assignment/4
  Demux/4 -> Bus Assignment/5
  Demux/5 -> Bus Assignment/6
  Demux/6 -> Bus Assignment/7
  Bus Assignment/1 -> Out1/1
  Demux/7 -> Bus Assignment/8
  Demux/8 -> Bus Assignment/9
  Demux/9 -> Bus Assignment/10

== system gtm_design/GTM_T2/TransportDelay/Transport Delay on Bus/BusDelay2 ==
  In1 : Inport
  Bus Assignment : BusAssignment  AssignedSignals=p_deg,q_deg,r_deg,Ax_g,Ay_g,Az_g
  Bus Selector1 : BusSelector  OutputSignals=p_deg,q_deg,r_deg,Ax_g,Ay_g,Az_g  OutputAsBus=on
  Bus to Vector : BusToVector
  Demux : Demux  Outputs=6
  TimeDelay with IC feedthrough : Subsystem  mask{TimeDelay=15e-3}
      mask prompts: TimeDelay "Time Delay (sec)"
      mask help:
      | Implements Continuous Time Transport Delay with initial
      | outputs set to feedthrough with no delay.
      |
      |   output = input;   for t<TimeDelay
      |   output = input(t-tdelay); for t>=TimeDelay
  Out1 : Outport
  wires:
  In1/1 -> Bus Assignment/1, Bus Selector1/1
  Bus Selector1/1 -> Bus to Vector/1
  Bus to Vector/1 -> TimeDelay with IC feedthrough/1(I)
  TimeDelay with IC feedthrough/1(O) -> Demux/1
  Demux/1 -> Bus Assignment/2
  Demux/2 -> Bus Assignment/3
  Demux/3 -> Bus Assignment/4
  Demux/4 -> Bus Assignment/5
  Demux/5 -> Bus Assignment/6
  Demux/6 -> Bus Assignment/7
  Bus Assignment/1 -> Out1/1

== system gtm_design/GTM_T2/TransportDelay/Transport Delay on Bus/BusDelay3 ==
  In1 : Inport
  Bus Assignment : BusAssignment  AssignedSignals=ELLOB,ELLIB,ELROB,ELRIB,AILL,AILR,RUDU,RUDL,FLAPLIB,FLAPLOB,FLAPRIB,FLAPROB
  Bus Selector1 : BusSelector  OutputSignals=ELLOB,ELLIB,ELROB,ELRIB,AILL,AILR,RUDU,RUDL,FLAPLIB,FLAPLOB,FLAPRIB,FLAPROB  OutputAsBus=on
  Bus to Vector : BusToVector
  Demux : Demux  Outputs=12
  TimeDelay with IC feedthrough : Subsystem  mask{TimeDelay=15e-3}
      mask prompts: TimeDelay "Time Delay (sec)"
      mask help:
      | Implements Continuous Time Transport Delay with initial
      | outputs set to feedthrough with no delay.
      |
      |   output = input;   for t<TimeDelay
      |   output = input(t-tdelay); for t>=TimeDelay
  Out1 : Outport
  wires:
  In1/1 -> Bus Assignment/1, Bus Selector1/1
  Bus Selector1/1 -> Bus to Vector/1
  Bus to Vector/1 -> TimeDelay with IC feedthrough/1(I)
  TimeDelay with IC feedthrough/1(O) -> Demux/1
  Bus Assignment/1 -> Out1/1
  Demux/1 -> Bus Assignment/2
  Demux/2 -> Bus Assignment/3
  Demux/3 -> Bus Assignment/4
  Demux/4 -> Bus Assignment/5
  Demux/5 -> Bus Assignment/6
  Demux/6 -> Bus Assignment/7
  Demux/7 -> Bus Assignment/8
  Demux/8 -> Bus Assignment/9
  Demux/9 -> Bus Assignment/10
  Demux/10 -> Bus Assignment/11
  Demux/11 -> Bus Assignment/12
  Demux/12 -> Bus Assignment/13

== system gtm_design/GTM_T2/TransportDelay/Transport Delay on Bus/BusDelay4 ==
  In1 : Inport
  Bus Assignment : BusAssignment  AssignedSignals=RPML,PUMPVL,RPMR,PUMPVR
  Bus Selector1 : BusSelector  OutputSignals=RPML,PUMPVL,RPMR,PUMPVR  OutputAsBus=on
  Bus to Vector : BusToVector
  Demux : Demux
  TimeDelay with IC feedthrough : Subsystem  mask{TimeDelay=15e-3}
      mask prompts: TimeDelay "Time Delay (sec)"
      mask help:
      | Implements Continuous Time Transport Delay with initial
      | outputs set to feedthrough with no delay.
      |
      |   output = input;   for t<TimeDelay
      |   output = input(t-tdelay); for t>=TimeDelay
  Out1 : Outport
  wires:
  In1/1 -> Bus Assignment/1, Bus Selector1/1
  Bus Selector1/1 -> Bus to Vector/1
  Bus to Vector/1 -> TimeDelay with IC feedthrough/1(I)
  TimeDelay with IC feedthrough/1(O) -> Demux/1
  Demux/1 -> Bus Assignment/2
  Demux/2 -> Bus Assignment/3
  Demux/3 -> Bus Assignment/4
  Demux/4 -> Bus Assignment/5
  Bus Assignment/1 -> Out1/1

== system gtm_design/GTM_T2/TransportDelay/Transport Delay on Bus1/BusDelay ==
  In1 : Inport
  Bus Assignment : BusAssignment  AssignedSignals=THROTLC,THROTRC,ELLOBC,ELLIBC,ELROBC,ELRIBC,AILLC,AILRC,RUDUPC,RUDLOC,SPLLIBC,SPLLOBC,SPLRIBC,SPLROBC,FLAPLC,MORPHLC,FLAPRC,MORPHRC,GEARC,BRAKEC,STEERC
  Bus Selector1 : BusSelector  OutputSignals=THROTLC,THROTRC,ELLOBC,ELLIBC,ELROBC,ELRIBC,AILLC,AILRC,RUDUPC,RUDLOC,SPLLIBC,SPLLOBC,SPLRIBC,SPLROBC,FLAPLC,MORPHLC,FLAPRC,MORPHRC,GEARC,BRAKEC,STEERC  OutputAsBus=on
  Bus to Vector : BusToVector
  Demux : Demux  Outputs=21
  Transport Delay : TransportDelay  DelayTime=5e-3
      settings: AttributesFormatString=%<DelayTime>
  Out1 : Outport
  wires:
  In1/1 -> Bus Assignment/1, Bus Selector1/1
  Bus Selector1/1 -> Bus to Vector/1
  Bus to Vector/1 -> Transport Delay/1
  Transport Delay/1 -> Demux/1
  Demux/1 -> Bus Assignment/2
  Demux/2 -> Bus Assignment/3
  Demux/3 -> Bus Assignment/4
  Demux/4 -> Bus Assignment/5
  Demux/5 -> Bus Assignment/6
  Demux/6 -> Bus Assignment/7
  Bus Assignment/1 -> Out1/1
  Demux/7 -> Bus Assignment/8
  Demux/8 -> Bus Assignment/9
  Demux/9 -> Bus Assignment/10
  Demux/10 -> Bus Assignment/11
  Demux/11 -> Bus Assignment/12
  Demux/12 -> Bus Assignment/13
  Demux/13 -> Bus Assignment/14
  Demux/14 -> Bus Assignment/15
  Demux/15 -> Bus Assignment/16
  Demux/16 -> Bus Assignment/17
  Demux/17 -> Bus Assignment/18
  Demux/18 -> Bus Assignment/19
  Demux/19 -> Bus Assignment/20
  Demux/20 -> Bus Assignment/21
  Demux/21 -> Bus Assignment/22

== system gtm_design/Guidance/Orbit Following/Subsystem1/Map 0_1 ==
  I : Inport
  Constant : Constant  Value=2*pi
  Constant1 : Constant  Value=0
  Gain : Gain  Gain=180/pi
  Sum : Sum  Inputs=|++
  ifnegadd2pi : Switch
  O : Outport
  wires:
  Gain/1 -> O/1
  Constant1/1 -> ifnegadd2pi/1
  Constant/1 -> ifnegadd2pi/3
  ifnegadd2pi/1 -> Sum/2
  Sum/1 -> Gain/1
  I/1 -> ifnegadd2pi/2, Sum/1

== system gtm_design/Guidance/Orbit Following/Subsystem1/VecNorm ==
  I : Inport
  Math Function2 : Math  Operator=sqrt  SignedPower=on  SaturateOnIntegerOverflow=on
  Product : Product  RndMeth=Zero
  Sum of Elements : Sum  Inputs=+
  O : Outport
  wires:
  Math Function2/1 -> O/1
  I/1 -> Product/1, Product/2
  Product/1 -> Sum of Elements/1
  Sum of Elements/1 -> Math Function2/1

== system gtm_design/Guidance/Waypoint Following/Subsystem1/Map 0_1 ==
  I : Inport
  Constant : Constant  Value=2*pi
  Constant1 : Constant  Value=0
  Gain : Gain  Gain=180/pi
  Sum : Sum  Inputs=|++
  ifnegadd2pi : Switch
  O : Outport
  wires:
  I/1 -> Sum/1, ifnegadd2pi/2
  Sum/1 -> Gain/1
  ifnegadd2pi/1 -> Sum/2
  Constant/1 -> ifnegadd2pi/3
  Constant1/1 -> ifnegadd2pi/1
  Gain/1 -> O/1

== system gtm_design/Guidance/Waypoint Following/Subsystem1/VecNorm ==
  I : Inport
  Math Function2 : Math  Operator=sqrt  SignedPower=on  SaturateOnIntegerOverflow=on
  Product : Product  RndMeth=Zero
  Sum of Elements : Sum  Inputs=+
  O : Outport
  wires:
  Sum of Elements/1 -> Math Function2/1
  Product/1 -> Sum of Elements/1
  I/1 -> Product/2, Product/1
  Math Function2/1 -> O/1

== system gtm_design/Control/Controller/Control Algorithm/Lateral-Directional Controller/Full State ==
  feedback : Inport
  Bus Selector : BusSelector  OutputSignals=AirData.beta_deg,MAG3.p_deg,MAG3.r_deg,MIDG.phi_deg
  Degrees to Radians{,1..2,6} (4 alike) : simulink_extras/Transformations/Degrees to Radians
  Mux : Mux
  bet_deg : Scope
  p_deg : Scope
  phi_deg : Scope
  r_deg : Scope
  x : Outport
  wires:
  Mux/1 -> x/1
  Degrees to Radians2/1 -> Mux/1  "bet_rad"
  Degrees to Radians6/1 -> Mux/4  "phi_rad"
  Degrees to Radians/1 -> Mux/2  "p_rad"
  Degrees to Radians1/1 -> Mux/3  "r_rad"
  Bus Selector/4 -> phi_deg/1, Degrees to Radians6/1  "<phi_deg>"
  Bus Selector/3 -> r_deg/1, Degrees to Radians1/1  "<r_deg>"
  Bus Selector/2 -> Degrees to Radians/1, p_deg/1  "<p_deg>"
  Bus Selector/1 -> Degrees to Radians2/1, bet_deg/1  "<beta_deg>"
  feedback/1 -> Bus Selector/1
